simulink model "ArmReflexGUI"  (R2025a)
settings: Solver=ode45  StartTime=0.0  StopTime=10  FixedStep=0.002  RelTol=1e-3
PreLoadFcn:
  | % --- elbow model ---
  | I_el  = 0.06;      % kg*m^2 forearm+cup inertia about elbow
  | b_el  = 2;         % N*m*s/rad damping
  | g     = 9.81;        % m/s^2
  | m_arm = 1.5;         % kg forearm mass
  | Lac   = 0.15;        % m forearm COM distance from elbow
  | Lcup  = 0.3;        % m cup distance from elbow
  | pourRate = 0.0625;   % kg/s beer pour (0.5 kg over 8 s)
  | % --- BPAs (real Festo 20 mm equations) ---
  | Pmax  = 620;         % kPa supply pressure
  | tauAct = 150;      % ms activation
  | L_hold = 0.185;      % m biceps length at level hold
  | c_len = 0.02;      % m biceps length change per rad sag (series compliance)
  | r_bi = 0.04;        % m biceps moment arm
  | L_hold_t = 0.185;   % m triceps length at level hold
  | c_len_t = 0.005;    % m triceps length change per rad sag
  | r_tri = 0.01;       % m triceps moment arm
  | A_bi0 = 0.3923778403;       % biceps activation holding the EMPTY cup (startup equilibrium)
  | A_tri0 = 0.4;      % triceps baseline co-contraction
  | % --- reflex ---
  | desc_bi  = 3.69618892;   % nA descending drive (empty-cup equilibrium)
  | desc_tri = 3.7;  % nA descending drive
  | sagN   = 3.333333333;      % normalize sag rad -> spindle input (~0.3 rad full span)
  | kReflex = 1;         % set 0 in runner to disable reflex synapses
libraries: SNS_Library x20, simulink x1
Description:
  | GUI-built stretch, force, and reciprocal feedback from the biceps and triceps sides, coupled to a pneumatic elbow resisting an increasing cup load.
settings Model: Creator=Ben Bolen  LastModifiedBy=Ben Bolen

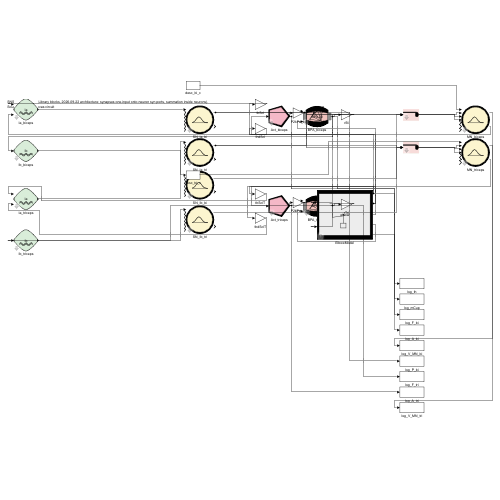
[thumbnail: Simulink's stored preview of the top-level diagram]
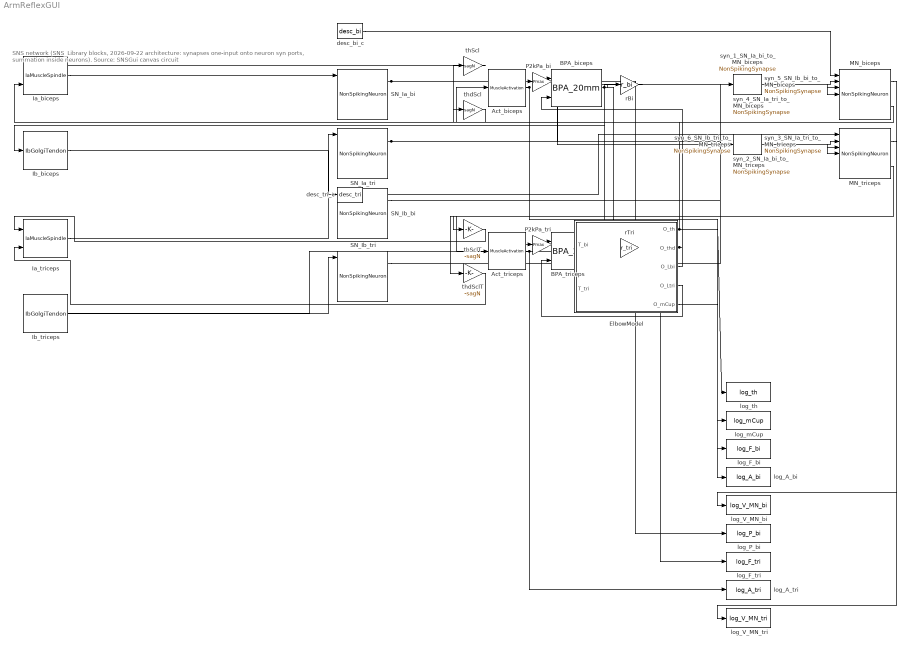
== system ArmReflexGUI ==
  note: SNS network (SNS_Library blocks, 2026-09-22 architecture: synapses one-input onto neuron syn ports, summation inside neurons).
      | Source: SNSGui canvas circuit
  Act_biceps : SNS_Library/MuscleActivation  tauAct=tauAct  A0=A_bi0
  Act_triceps : SNS_Library/MuscleActivation  tauAct=tauAct  A0=A_tri0
  BPA_biceps : SNS_Library/BPA_20mm  Rest=0.20  Kmax=0.165  TendonL=0  FittingL=0
  BPA_triceps : SNS_Library/BPA_20mm  Rest=0.20  Kmax=0.165  TendonL=0  FittingL=0
  ElbowModel : Subsystem  mask(SNS Elbow Model (1-DOF)){}
      mask help: 1-DOF elbow with cup: I*thdd = T_biceps - T_triceps - b*thd + T_grav, T_grav = (m_cup(t)*Lcup + m_arm*Lac)*g*cos(theta); beer pours at pourRate. Outputs: theta (sag, rad), thd, biceps length, triceps length, m_cup.
      mask Display:
      | patch([-1 1 1 -1], [-1 -1 1 1], [0 0 0]);
      | patch([-0.92 0.92 0.92 -0.92], [-0.84 -0.84 0.84 0.84], [0.93 0.93 0.93]);
      | color('black');
      | plot([-0.55 -0.45], [0.45 0.45]);
      | plot([-0.45 -0.45], [0.45 -0.10]);
      | plot([-0.45 -0.05], [-0.10 -0.05]);
      | plot([-0.05 -0.05], [-0.05 -0.35]);
      | patch(-0.05 + 0.08*cos(0.3927 + (0:0.0628:1.5708)), -0.05 + 0.08*sin(0.3927 + (0:0.0628:1.5708)), [1 1 1]);
      | patch(-0.05 + 0.05*cos(0.3927 + (0:0.0628:1.5708)), -0.05 + 0.05*sin(0.3927 + (0:0.0628:1.5708)), [0 0 0]);
      | plot([-0.15 0.05 0.05 -0.15 -0.15], [-0.35 -0.35 -0.55 -0.55 -0.35]);
      | disp('elbow');
  Ia_biceps : SNS_Library/IaMuscleSpindle  Imax=10  Wl=24  Wv=8
  Ia_triceps : SNS_Library/IaMuscleSpindle  Imax=10  Wl=24  Wv=8
  Ib_biceps : SNS_Library/IbGolgiTendon  Imax=10  Kf=0.008
  Ib_triceps : SNS_Library/IbGolgiTendon  Imax=10  Kf=0.008
  MN_biceps : SNS_Library/NonSpikingNeuron  Vrest=-52  Gm=0.5  Cm=5  Thr=-45  Slope=1
  MN_triceps : SNS_Library/NonSpikingNeuron  Vrest=-52  Gm=0.5  Cm=5  Thr=-45  Slope=1
  P2kPa_bi : Gain  Gain=Pmax
  P2kPa_tri : Gain  Gain=Pmax
  SN_Ia_bi : SNS_Library/NonSpikingNeuron  Vrest=-52  Gm=0.12  Cm=2  Thr=-55  Slope=1
  SN_Ia_tri : SNS_Library/NonSpikingNeuron  Vrest=-52  Gm=0.12  Cm=2  Thr=-55  Slope=1
  SN_Ib_bi : SNS_Library/NonSpikingNeuron  Vrest=-52  Gm=0.4  Cm=2  Thr=-55  Slope=1
  SN_Ib_tri : SNS_Library/NonSpikingNeuron  Vrest=-52  Gm=0.4  Cm=2  Thr=-55  Slope=1
  desc_bi_c : Constant  Value=desc_bi
  desc_tri_c : Constant  Value=desc_tri
  log_A_bi : ToWorkspace  VariableName=log_A_bi  SaveFormat=Timeseries  SampleTime=-1
  log_A_tri : ToWorkspace  VariableName=log_A_tri  SaveFormat=Timeseries  SampleTime=-1
  log_F_bi : ToWorkspace  VariableName=log_F_bi  SaveFormat=Timeseries  SampleTime=-1
  log_F_tri : ToWorkspace  VariableName=log_F_tri  SaveFormat=Timeseries  SampleTime=-1
  log_P_bi : ToWorkspace  VariableName=log_P_bi  SaveFormat=Timeseries  SampleTime=-1
  log_V_MN_bi : ToWorkspace  VariableName=log_V_MN_bi  SaveFormat=Timeseries  SampleTime=-1
  log_V_MN_tri : ToWorkspace  VariableName=log_V_MN_tri  SaveFormat=Timeseries  SampleTime=-1
  log_mCup : ToWorkspace  VariableName=log_mCup  SaveFormat=Timeseries  SampleTime=-1
  log_th : ToWorkspace  VariableName=log_th  SaveFormat=Timeseries  SampleTime=-1
  rBi : Gain  Gain=r_bi
  rTri : Gain  Gain=r_tri
  syn_1_SN_Ia_bi_to_MN_biceps : SNS_Library/NonSpikingSynapse  gmax=0.0005  Esyn=0  ThrPre=-45  SlopePre=0.5
  syn_2_SN_Ia_bi_to_MN_triceps : SNS_Library/NonSpikingSynapse  gmax=0.0025  Esyn=-72  ThrPre=-45  SlopePre=0.5
  syn_3_SN_Ia_tri_to_MN_triceps : SNS_Library/NonSpikingSynapse  gmax=0.001  Esyn=0  ThrPre=-45  SlopePre=0.5
  syn_4_SN_Ia_tri_to_MN_biceps : SNS_Library/NonSpikingSynapse  gmax=0.0008  Esyn=-72  ThrPre=-45  SlopePre=0.5
  syn_5_SN_Ib_bi_to_MN_biceps : SNS_Library/NonSpikingSynapse  gmax=0.0006  Esyn=-72  ThrPre=-45  SlopePre=0.5
  syn_6_SN_Ib_tri_to_MN_triceps : SNS_Library/NonSpikingSynapse  gmax=0.0004  Esyn=-72  ThrPre=-45  SlopePre=0.5
  thScl : Gain  Gain=sagN
  thSclT : Gain  Gain=-sagN
  thdScl : Gain  Gain=sagN
  thdSclT : Gain  Gain=-sagN
  wires:
  syn_1_SN_Ia_bi_to_MN_biceps/1 -> MN_biceps/2
  syn_4_SN_Ia_tri_to_MN_biceps/1 -> MN_biceps/3
  syn_5_SN_Ib_bi_to_MN_biceps/1 -> MN_biceps/4
  syn_2_SN_Ia_bi_to_MN_triceps/1 -> MN_triceps/2
  syn_3_SN_Ia_tri_to_MN_triceps/1 -> MN_triceps/3
  syn_6_SN_Ib_tri_to_MN_triceps/1 -> MN_triceps/4
  SN_Ia_bi/1 -> syn_1_SN_Ia_bi_to_MN_biceps/1, syn_2_SN_Ia_bi_to_MN_triceps/1
  SN_Ia_tri/1 -> syn_3_SN_Ia_tri_to_MN_triceps/1, syn_4_SN_Ia_tri_to_MN_biceps/1
  SN_Ib_bi/1 -> syn_5_SN_Ib_bi_to_MN_biceps/1
  SN_Ib_tri/1 -> syn_6_SN_Ib_tri_to_MN_triceps/1
  MN_biceps/2 -> Act_biceps/1
  MN_triceps/2 -> Act_triceps/1
  P2kPa_bi/1 -> BPA_biceps/1, log_P_bi/1
  ElbowModel/3(O_Lbi) -> BPA_biceps/2
  P2kPa_tri/1 -> BPA_triceps/1
  ElbowModel/4(O_Ltri) -> BPA_triceps/2
  rBi/1 -> ElbowModel/1(T_bi)
  rTri/1 -> ElbowModel/2(T_tri)
  thScl/1 -> Ia_biceps/1
  thdScl/1 -> Ia_biceps/2
  thSclT/1 -> Ia_triceps/1
  thdSclT/1 -> Ia_triceps/2
  BPA_biceps/1 -> Ib_biceps/1, log_F_bi/1, rBi/1
  BPA_triceps/1 -> Ib_triceps/1, log_F_tri/1, rTri/1
  desc_bi_c/1 -> MN_biceps/1
  desc_tri_c/1 -> MN_triceps/1
  Act_biceps/1 -> P2kPa_bi/1, log_A_bi/1
  Act_triceps/1 -> P2kPa_tri/1, log_A_tri/1
  Ia_biceps/1 -> SN_Ia_bi/1
  Ia_triceps/1 -> SN_Ia_tri/1
  Ib_biceps/1 -> SN_Ib_bi/1
  Ib_triceps/1 -> SN_Ib_tri/1
  MN_biceps/1 -> log_V_MN_bi/1
  MN_triceps/1 -> log_V_MN_tri/1
  ElbowModel/5(O_mCup) -> log_mCup/1
  ElbowModel/1(O_th) -> log_th/1, thScl/1, thSclT/1
  ElbowModel/2(O_thd) -> thdScl/1, thdSclT/1

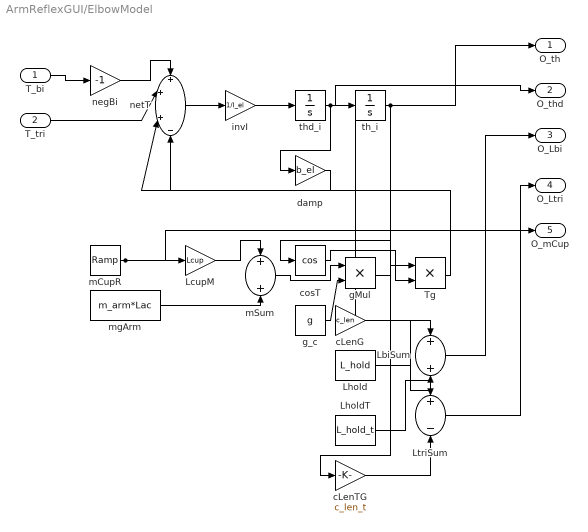
== system ArmReflexGUI/ElbowModel ==
  T_bi : Inport
  T_tri : Inport  Port=2
  LbiSum : Sum
  LcupM : Gain  Gain=Lcup
  Lhold : Constant  Value=L_hold
  LholdT : Constant  Value=L_hold_t
  LtriSum : Sum  Inputs=+-
  Tg : Product
  cLenG : Gain  Gain=c_len
  cLenTG : Gain  Gain=c_len_t
  cosT : Trigonometry  Operator=cos
  damp : Gain  Gain=b_el
  gMul : Product
  g_c : Constant  Value=g
  invI : Gain  Gain=1/I_el
  mCupR : simulink/Sources/Ramp  slope=pourRate  start=0  InitialOutput=0
  mSum : Sum
  mgArm : Constant  Value=m_arm*Lac
  negBi : Gain  Gain=-1
  netT : Sum  Inputs=+++-
  th_i : Integrator
  thd_i : Integrator
  O_th : Outport
  O_thd : Outport  Port=2
  O_Lbi : Outport  Port=3
  O_Ltri : Outport  Port=4
  O_mCup : Outport  Port=5
  wires:
  LtriSum/1 -> O_Ltri/1
  cLenTG/1 -> LtriSum/2
  LholdT/1 -> LtriSum/1
  LbiSum/1 -> O_Lbi/1
  cLenG/1 -> LbiSum/2
  Lhold/1 -> LbiSum/1
  Tg/1 -> netT/3
  cosT/1 -> Tg/2
  gMul/1 -> Tg/1
  g_c/1 -> gMul/2
  mSum/1 -> gMul/1
  mgArm/1 -> mSum/2
  LcupM/1 -> mSum/1
  mCupR/1 -> O_mCup/1, LcupM/1
  th_i/1 -> cLenTG/1, cLenG/1, O_th/1, cosT/1
  damp/1 -> netT/4
  thd_i/1 -> O_thd/1, damp/1, th_i/1
  invI/1 -> thd_i/1
  netT/1 -> invI/1
  negBi/1 -> netT/1
  T_tri/1 -> netT/2
  T_bi/1 -> negBi/1
